simulink model "model_new_visual"  (R2023a)
settings: Solver=VariableStepAuto  StartTime=0.0  StopTime=3  RelTol=1e-3
model workspace: external: MATLAB File model_new_DataFile.m (data not in the file)
values from neighbouring files (symbols this model uses):
  smiData = struct    [model_new_DataFile.m]
undefined symbols (not defined in the file or in its folder): _, ____, ____16, ____19, ____20, ____3, ____4, ____4X6X3, ____6, ____6X10X3, ____7X11X2, ______, ______1, ______2, ______3_________________________, _______1_________________________2_________________________________航发支架总装, ________, ________1, ________20__1____6, ________6, _________, __________, __________2, __________40160, __________6x16x5, ____________, ____________2, ____________3X1, ______________, ______________1X5, __________________, ___________________, ____________________20__26____4, ____________________25__25____5, __________________SULERCH, ______________A, __________A, __________B, ______A__6, _X2_4E1D6746_X0_, _X2_652F64915EA7_X0_, _X2_7535673A5B8988C5677F_X0_, _X2_8F74627F677F_X0_, _航发支架总装, _默认_sldprt, A25, a__________100, BZ, C, CONNECTOR_5MMCLOSED2PIN_MALE_1, D1, DIP_SWITCH_8PIN_VIC2_1, DYJN, EC, EE, FUS606_REF_1, GE4C, IPOS__________, LAF30, M3________ ... (+34)
libraries: sm_lib x987, nesl_utility x6, simulink x4
(part 18 of 18)

== system model_new_visual/x__25_07_22_V1_STEP_1_RIGID/Subsystem/x__25_07_22_V1_STEP_1_RIGID1/CL3J_EC503_3D_25_07_22_V1_STEP_1_RIGID/PCB_ASM_4_ASM25_07_22_V1_STEP_1_RIGID/x5PIN_MINIUSB_SOCKET_1_1_125_07_22_V1_STEP_1_RIGID ==
  ReferenceFrame : sm_lib/Frames and Transforms/Reference Frame
  Solid : sm_lib/Body Elements/File Solid  ExtGeomFileName=5PIN_MINIUSB_SOCKET_1_1_1(25.07.22)-V1.STEP_默认_sldprt.STEP  UnitType=FromFile  ExtGeomFileUnits=m  StepReaderType=HEX  ExportConvexHullGeometry=off  InertiaType=Custom  Mass=smiData.Solid(76).mass  MassUnits=kg  CenterOfMass=smiData.Solid(76).CoM  CenterOfMassUnits=mm  MomentsOfInertia=smiData.Solid(76).MoI  MomentsOfInertiaUnits=kg*mm^2  ProductsOfInertia=smiData.Solid(76).PoI  ProductsOfInertiaUnits=kg*mm^2  BasedOnType=DensityFromFile  Density=1000  DensityUnits=kg/m^3  DoExposeReferenceFrame=on  SerializedFrames=<Frames/>  GraphicType=FromGeometry  MarkerShape=Sphere  MarkerSize=10  GraphicVisPropType=SimpleVisualProperties  GraphicDiffuseColor=smiData.Solid(76).color  GraphicSpecularColor=[0.5 0.5 0.5 1.0]  GraphicAmbientColor=[0.15 0.15 0.15 1.0]  GraphicEmissiveColor=[0.0 0.0 0.0 1.0]  GraphicShininess=75  GraphicOpacity=smiData.Solid(76).opacity
  F : PMIOPort  Side=Left
  connections:
  Solid/RConn1 -- ReferenceFrame/RConn1 -- F/RConn1

== system model_new_visual/x__25_07_22_V1_STEP_1_RIGID/Subsystem/x__25_07_22_V1_STEP_1_RIGID1/CL3J_EC503_3D_25_07_22_V1_STEP_1_RIGID/PCB_ASM_4_ASM25_07_22_V1_STEP_1_RIGID/FCI_USB_ANY_1_ASM25_07_22_V1_STEP_1_RIGID/MANIFOLD_SOLID_BREP_6679525_07_22_V1_STEP_1_RIGID ==
  ReferenceFrame : sm_lib/Frames and Transforms/Reference Frame
  Solid : sm_lib/Body Elements/File Solid  ExtGeomFileName=MANIFOLD_SOLID_BREP_66795(25.07.22)-V1.STEP_默认_sldprt.STEP  UnitType=FromFile  ExtGeomFileUnits=m  StepReaderType=HEX  ExportConvexHullGeometry=off  InertiaType=Custom  Mass=smiData.Solid(79).mass  MassUnits=kg  CenterOfMass=smiData.Solid(79).CoM  CenterOfMassUnits=mm  MomentsOfInertia=smiData.Solid(79).MoI  MomentsOfInertiaUnits=kg*mm^2  ProductsOfInertia=smiData.Solid(79).PoI  ProductsOfInertiaUnits=kg*mm^2  BasedOnType=DensityFromFile  Density=1000  DensityUnits=kg/m^3  DoExposeReferenceFrame=on  SerializedFrames=<Frames/>  GraphicType=FromGeometry  MarkerShape=Sphere  MarkerSize=10  GraphicVisPropType=SimpleVisualProperties  GraphicDiffuseColor=smiData.Solid(79).color  GraphicSpecularColor=[0.5 0.5 0.5 1.0]  GraphicAmbientColor=[0.15 0.15 0.15 1.0]  GraphicEmissiveColor=[0.0 0.0 0.0 1.0]  GraphicShininess=75  GraphicOpacity=smiData.Solid(79).opacity
  F : PMIOPort  Side=Left
  connections:
  Solid/RConn1 -- ReferenceFrame/RConn1 -- F/RConn1

== system model_new_visual/x__25_07_22_V1_STEP_1_RIGID/Subsystem/x__25_07_22_V1_STEP_1_RIGID1/CL3J_EC503_3D_25_07_22_V1_STEP_1_RIGID/PCB_ASM_4_ASM25_07_22_V1_STEP_1_RIGID/FCI_USB_ANY_1_ASM25_07_22_V1_STEP_1_RIGID/MANIFOLD_SOLID_BREP_6688325_07_22_V1_STEP_1_RIGID ==
  ReferenceFrame : sm_lib/Frames and Transforms/Reference Frame
  Solid : sm_lib/Body Elements/File Solid  ExtGeomFileName=MANIFOLD_SOLID_BREP_66883(25.07.22)-V1.STEP_默认_sldprt.STEP  UnitType=FromFile  ExtGeomFileUnits=m  StepReaderType=HEX  ExportConvexHullGeometry=off  InertiaType=Custom  Mass=smiData.Solid(78).mass  MassUnits=kg  CenterOfMass=smiData.Solid(78).CoM  CenterOfMassUnits=mm  MomentsOfInertia=smiData.Solid(78).MoI  MomentsOfInertiaUnits=kg*mm^2  ProductsOfInertia=smiData.Solid(78).PoI  ProductsOfInertiaUnits=kg*mm^2  BasedOnType=DensityFromFile  Density=1000  DensityUnits=kg/m^3  DoExposeReferenceFrame=on  SerializedFrames=<Frames/>  GraphicType=FromGeometry  MarkerShape=Sphere  MarkerSize=10  GraphicVisPropType=SimpleVisualProperties  GraphicDiffuseColor=smiData.Solid(78).color  GraphicSpecularColor=[0.5 0.5 0.5 1.0]  GraphicAmbientColor=[0.15 0.15 0.15 1.0]  GraphicEmissiveColor=[0.0 0.0 0.0 1.0]  GraphicShininess=75  GraphicOpacity=smiData.Solid(78).opacity
  F : PMIOPort  Side=Left
  connections:
  Solid/RConn1 -- ReferenceFrame/RConn1 -- F/RConn1

== system model_new_visual/x__25_07_22_V1_STEP_1_RIGID/Subsystem/x__25_07_22_V1_STEP_1_RIGID1/CL3J_EC503_3D_25_07_22_V1_STEP_1_RIGID/PCB_ASM_4_ASM25_07_22_V1_STEP_1_RIGID/x15EDGRHB_THR_3_5_10_1_ASM25_07_22_V1_STEP_1_RIGID/MANIFOLD_SOLID_BREP_11810025_07_22_V1_STEP_1_RIGID ==
  ReferenceFrame : sm_lib/Frames and Transforms/Reference Frame
  Solid : sm_lib/Body Elements/File Solid  ExtGeomFileName=MANIFOLD_SOLID_BREP_118100(25.07.22)-V1.STEP_默认_sldprt.STEP  UnitType=FromFile  ExtGeomFileUnits=m  StepReaderType=HEX  ExportConvexHullGeometry=off  InertiaType=Custom  Mass=smiData.Solid(82).mass  MassUnits=kg  CenterOfMass=smiData.Solid(82).CoM  CenterOfMassUnits=mm  MomentsOfInertia=smiData.Solid(82).MoI  MomentsOfInertiaUnits=kg*mm^2  ProductsOfInertia=smiData.Solid(82).PoI  ProductsOfInertiaUnits=kg*mm^2  BasedOnType=DensityFromFile  Density=1000  DensityUnits=kg/m^3  DoExposeReferenceFrame=on  SerializedFrames=<Frames/>  GraphicType=FromGeometry  MarkerShape=Sphere  MarkerSize=10  GraphicVisPropType=SimpleVisualProperties  GraphicDiffuseColor=smiData.Solid(82).color  GraphicSpecularColor=[0.5 0.5 0.5 1.0]  GraphicAmbientColor=[0.15 0.15 0.15 1.0]  GraphicEmissiveColor=[0.0 0.0 0.0 1.0]  GraphicShininess=75  GraphicOpacity=smiData.Solid(82).opacity
  F : PMIOPort  Side=Left
  connections:
  Solid/RConn1 -- ReferenceFrame/RConn1 -- F/RConn1

== system model_new_visual/x__25_07_22_V1_STEP_1_RIGID/Subsystem/x__25_07_22_V1_STEP_1_RIGID1/CL3J_EC503_3D_25_07_22_V1_STEP_1_RIGID/PCB_ASM_4_ASM25_07_22_V1_STEP_1_RIGID/x15EDGRHB_THR_3_5_10_1_ASM25_07_22_V1_STEP_1_RIGID/MANIFOLD_SOLID_BREP_11834725_07_22_V1_STEP_1_RIGID ==
  ReferenceFrame : sm_lib/Frames and Transforms/Reference Frame
  Solid : sm_lib/Body Elements/File Solid  ExtGeomFileName=MANIFOLD_SOLID_BREP_118347(25.07.22)-V1.STEP_默认_sldprt.STEP  UnitType=FromFile  ExtGeomFileUnits=m  StepReaderType=HEX  ExportConvexHullGeometry=off  InertiaType=Custom  Mass=smiData.Solid(83).mass  MassUnits=kg  CenterOfMass=smiData.Solid(83).CoM  CenterOfMassUnits=mm  MomentsOfInertia=smiData.Solid(83).MoI  MomentsOfInertiaUnits=kg*mm^2  ProductsOfInertia=smiData.Solid(83).PoI  ProductsOfInertiaUnits=kg*mm^2  BasedOnType=DensityFromFile  Density=1000  DensityUnits=kg/m^3  DoExposeReferenceFrame=on  SerializedFrames=<Frames/>  GraphicType=FromGeometry  MarkerShape=Sphere  MarkerSize=10  GraphicVisPropType=SimpleVisualProperties  GraphicDiffuseColor=smiData.Solid(83).color  GraphicSpecularColor=[0.5 0.5 0.5 1.0]  GraphicAmbientColor=[0.15 0.15 0.15 1.0]  GraphicEmissiveColor=[0.0 0.0 0.0 1.0]  GraphicShininess=75  GraphicOpacity=smiData.Solid(83).opacity
  F : PMIOPort  Side=Left
  connections:
  Solid/RConn1 -- ReferenceFrame/RConn1 -- F/RConn1

== system model_new_visual/x__25_07_22_V1_STEP_1_RIGID/Subsystem/x__25_07_22_V1_STEP_1_RIGID1/CL3J_EC503_3D_25_07_22_V1_STEP_1_RIGID/PCB_ASM_4_ASM25_07_22_V1_STEP_1_RIGID/x15EDGRHB_THR_3_5_10_1_ASM25_07_22_V1_STEP_1_RIGID/MANIFOLD_SOLID_BREP_11859425_07_22_V1_STEP_1_RIGID ==
  ReferenceFrame : sm_lib/Frames and Transforms/Reference Frame
  Solid : sm_lib/Body Elements/File Solid  ExtGeomFileName=MANIFOLD_SOLID_BREP_118594(25.07.22)-V1.STEP_默认_sldprt.STEP  UnitType=FromFile  ExtGeomFileUnits=m  StepReaderType=HEX  ExportConvexHullGeometry=off  InertiaType=Custom  Mass=smiData.Solid(85).mass  MassUnits=kg  CenterOfMass=smiData.Solid(85).CoM  CenterOfMassUnits=mm  MomentsOfInertia=smiData.Solid(85).MoI  MomentsOfInertiaUnits=kg*mm^2  ProductsOfInertia=smiData.Solid(85).PoI  ProductsOfInertiaUnits=kg*mm^2  BasedOnType=DensityFromFile  Density=1000  DensityUnits=kg/m^3  DoExposeReferenceFrame=on  SerializedFrames=<Frames/>  GraphicType=FromGeometry  MarkerShape=Sphere  MarkerSize=10  GraphicVisPropType=SimpleVisualProperties  GraphicDiffuseColor=smiData.Solid(85).color  GraphicSpecularColor=[0.5 0.5 0.5 1.0]  GraphicAmbientColor=[0.15 0.15 0.15 1.0]  GraphicEmissiveColor=[0.0 0.0 0.0 1.0]  GraphicShininess=75  GraphicOpacity=smiData.Solid(85).opacity
  F : PMIOPort  Side=Left
  connections:
  Solid/RConn1 -- ReferenceFrame/RConn1 -- F/RConn1

== system model_new_visual/x__25_07_22_V1_STEP_1_RIGID/Subsystem/x__25_07_22_V1_STEP_1_RIGID1/CL3J_EC503_3D_25_07_22_V1_STEP_1_RIGID/PCB_ASM_4_ASM25_07_22_V1_STEP_1_RIGID/x15EDGRHB_THR_3_5_10_1_ASM25_07_22_V1_STEP_1_RIGID/MANIFOLD_SOLID_BREP_11884125_07_22_V1_STEP_1_RIGID ==
  ReferenceFrame : sm_lib/Frames and Transforms/Reference Frame
  Solid : sm_lib/Body Elements/File Solid  ExtGeomFileName=MANIFOLD_SOLID_BREP_118841(25.07.22)-V1.STEP_默认_sldprt.STEP  UnitType=FromFile  ExtGeomFileUnits=m  StepReaderType=HEX  ExportConvexHullGeometry=off  InertiaType=Custom  Mass=smiData.Solid(81).mass  MassUnits=kg  CenterOfMass=smiData.Solid(81).CoM  CenterOfMassUnits=mm  MomentsOfInertia=smiData.Solid(81).MoI  MomentsOfInertiaUnits=kg*mm^2  ProductsOfInertia=smiData.Solid(81).PoI  ProductsOfInertiaUnits=kg*mm^2  BasedOnType=DensityFromFile  Density=1000  DensityUnits=kg/m^3  DoExposeReferenceFrame=on  SerializedFrames=<Frames/>  GraphicType=FromGeometry  MarkerShape=Sphere  MarkerSize=10  GraphicVisPropType=SimpleVisualProperties  GraphicDiffuseColor=smiData.Solid(81).color  GraphicSpecularColor=[0.5 0.5 0.5 1.0]  GraphicAmbientColor=[0.15 0.15 0.15 1.0]  GraphicEmissiveColor=[0.0 0.0 0.0 1.0]  GraphicShininess=75  GraphicOpacity=smiData.Solid(81).opacity
  F : PMIOPort  Side=Left
  connections:
  Solid/RConn1 -- ReferenceFrame/RConn1 -- F/RConn1

== system model_new_visual/x__25_07_22_V1_STEP_1_RIGID/Subsystem/x__25_07_22_V1_STEP_1_RIGID1/CL3J_EC503_3D_25_07_22_V1_STEP_1_RIGID/PCB_ASM_4_ASM25_07_22_V1_STEP_1_RIGID/x15EDGRHB_THR_3_5_10_1_ASM25_07_22_V1_STEP_1_RIGID/MANIFOLD_SOLID_BREP_11908825_07_22_V1_STEP_1_RIGID ==
  ReferenceFrame : sm_lib/Frames and Transforms/Reference Frame
  Solid : sm_lib/Body Elements/File Solid  ExtGeomFileName=MANIFOLD_SOLID_BREP_119088(25.07.22)-V1.STEP_默认_sldprt.STEP  UnitType=FromFile  ExtGeomFileUnits=m  StepReaderType=HEX  ExportConvexHullGeometry=off  InertiaType=Custom  Mass=smiData.Solid(84).mass  MassUnits=kg  CenterOfMass=smiData.Solid(84).CoM  CenterOfMassUnits=mm  MomentsOfInertia=smiData.Solid(84).MoI  MomentsOfInertiaUnits=kg*mm^2  ProductsOfInertia=smiData.Solid(84).PoI  ProductsOfInertiaUnits=kg*mm^2  BasedOnType=DensityFromFile  Density=1000  DensityUnits=kg/m^3  DoExposeReferenceFrame=on  SerializedFrames=<Frames/>  GraphicType=FromGeometry  MarkerShape=Sphere  MarkerSize=10  GraphicVisPropType=SimpleVisualProperties  GraphicDiffuseColor=smiData.Solid(84).color  GraphicSpecularColor=[0.5 0.5 0.5 1.0]  GraphicAmbientColor=[0.15 0.15 0.15 1.0]  GraphicEmissiveColor=[0.0 0.0 0.0 1.0]  GraphicShininess=75  GraphicOpacity=smiData.Solid(84).opacity
  F : PMIOPort  Side=Left
  connections:
  Solid/RConn1 -- ReferenceFrame/RConn1 -- F/RConn1

== system model_new_visual/x__25_07_22_V1_STEP_1_RIGID/Subsystem/x__25_07_22_V1_STEP_1_RIGID1/CL3J_EC503_3D_25_07_22_V1_STEP_1_RIGID/PCB_ASM_4_ASM25_07_22_V1_STEP_1_RIGID/x15EDGRHB_THR_3_5_10_1_ASM25_07_22_V1_STEP_1_RIGID/MANIFOLD_SOLID_BREP_11933525_07_22_V1_STEP_1_RIGID ==
  ReferenceFrame : sm_lib/Frames and Transforms/Reference Frame
  Solid : sm_lib/Body Elements/File Solid  ExtGeomFileName=MANIFOLD_SOLID_BREP_119335(25.07.22)-V1.STEP_默认_sldprt.STEP  UnitType=FromFile  ExtGeomFileUnits=m  StepReaderType=HEX  ExportConvexHullGeometry=off  InertiaType=Custom  Mass=smiData.Solid(80).mass  MassUnits=kg  CenterOfMass=smiData.Solid(80).CoM  CenterOfMassUnits=mm  MomentsOfInertia=smiData.Solid(80).MoI  MomentsOfInertiaUnits=kg*mm^2  ProductsOfInertia=smiData.Solid(80).PoI  ProductsOfInertiaUnits=kg*mm^2  BasedOnType=DensityFromFile  Density=1000  DensityUnits=kg/m^3  DoExposeReferenceFrame=on  SerializedFrames=<Frames/>  GraphicType=FromGeometry  MarkerShape=Sphere  MarkerSize=10  GraphicVisPropType=SimpleVisualProperties  GraphicDiffuseColor=smiData.Solid(80).color  GraphicSpecularColor=[0.5 0.5 0.5 1.0]  GraphicAmbientColor=[0.15 0.15 0.15 1.0]  GraphicEmissiveColor=[0.0 0.0 0.0 1.0]  GraphicShininess=75  GraphicOpacity=smiData.Solid(80).opacity
  F : PMIOPort  Side=Left
  connections:
  Solid/RConn1 -- ReferenceFrame/RConn1 -- F/RConn1

== system model_new_visual/x__25_07_22_V1_STEP_1_RIGID/Subsystem/x__25_07_22_V1_STEP_1_RIGID1/CL3J_EC503_3D_25_07_22_V1_STEP_1_RIGID/PCB_ASM_4_ASM25_07_22_V1_STEP_1_RIGID/x15EDGRHB_THR_3_5_10_1_ASM25_07_22_V1_STEP_1_RIGID/MANIFOLD_SOLID_BREP_11958225_07_22_V1_STEP_1_RIGID ==
  ReferenceFrame : sm_lib/Frames and Transforms/Reference Frame
  Solid : sm_lib/Body Elements/File Solid  ExtGeomFileName=MANIFOLD_SOLID_BREP_119582(25.07.22)-V1.STEP_默认_sldprt.STEP  UnitType=FromFile  ExtGeomFileUnits=m  StepReaderType=HEX  ExportConvexHullGeometry=off  InertiaType=Custom  Mass=smiData.Solid(90).mass  MassUnits=kg  CenterOfMass=smiData.Solid(90).CoM  CenterOfMassUnits=mm  MomentsOfInertia=smiData.Solid(90).MoI  MomentsOfInertiaUnits=kg*mm^2  ProductsOfInertia=smiData.Solid(90).PoI  ProductsOfInertiaUnits=kg*mm^2  BasedOnType=DensityFromFile  Density=1000  DensityUnits=kg/m^3  DoExposeReferenceFrame=on  SerializedFrames=<Frames/>  GraphicType=FromGeometry  MarkerShape=Sphere  MarkerSize=10  GraphicVisPropType=SimpleVisualProperties  GraphicDiffuseColor=smiData.Solid(90).color  GraphicSpecularColor=[0.5 0.5 0.5 1.0]  GraphicAmbientColor=[0.15 0.15 0.15 1.0]  GraphicEmissiveColor=[0.0 0.0 0.0 1.0]  GraphicShininess=75  GraphicOpacity=smiData.Solid(90).opacity
  F : PMIOPort  Side=Left
  connections:
  Solid/RConn1 -- ReferenceFrame/RConn1 -- F/RConn1

== system model_new_visual/x__25_07_22_V1_STEP_1_RIGID/Subsystem/x__25_07_22_V1_STEP_1_RIGID1/CL3J_EC503_3D_25_07_22_V1_STEP_1_RIGID/PCB_ASM_4_ASM25_07_22_V1_STEP_1_RIGID/x15EDGRHB_THR_3_5_10_1_ASM25_07_22_V1_STEP_1_RIGID/MANIFOLD_SOLID_BREP_11982925_07_22_V1_STEP_1_RIGID ==
  ReferenceFrame : sm_lib/Frames and Transforms/Reference Frame
  Solid : sm_lib/Body Elements/File Solid  ExtGeomFileName=MANIFOLD_SOLID_BREP_119829(25.07.22)-V1.STEP_默认_sldprt.STEP  UnitType=FromFile  ExtGeomFileUnits=m  StepReaderType=HEX  ExportConvexHullGeometry=off  InertiaType=Custom  Mass=smiData.Solid(89).mass  MassUnits=kg  CenterOfMass=smiData.Solid(89).CoM  CenterOfMassUnits=mm  MomentsOfInertia=smiData.Solid(89).MoI  MomentsOfInertiaUnits=kg*mm^2  ProductsOfInertia=smiData.Solid(89).PoI  ProductsOfInertiaUnits=kg*mm^2  BasedOnType=DensityFromFile  Density=1000  DensityUnits=kg/m^3  DoExposeReferenceFrame=on  SerializedFrames=<Frames/>  GraphicType=FromGeometry  MarkerShape=Sphere  MarkerSize=10  GraphicVisPropType=SimpleVisualProperties  GraphicDiffuseColor=smiData.Solid(89).color  GraphicSpecularColor=[0.5 0.5 0.5 1.0]  GraphicAmbientColor=[0.15 0.15 0.15 1.0]  GraphicEmissiveColor=[0.0 0.0 0.0 1.0]  GraphicShininess=75  GraphicOpacity=smiData.Solid(89).opacity
  F : PMIOPort  Side=Left
  connections:
  Solid/RConn1 -- ReferenceFrame/RConn1 -- F/RConn1

== system model_new_visual/x__25_07_22_V1_STEP_1_RIGID/Subsystem/x__25_07_22_V1_STEP_1_RIGID1/CL3J_EC503_3D_25_07_22_V1_STEP_1_RIGID/PCB_ASM_4_ASM25_07_22_V1_STEP_1_RIGID/x15EDGRHB_THR_3_5_10_1_ASM25_07_22_V1_STEP_1_RIGID/MANIFOLD_SOLID_BREP_12007625_07_22_V1_STEP_1_RIGID ==
  ReferenceFrame : sm_lib/Frames and Transforms/Reference Frame
  Solid : sm_lib/Body Elements/File Solid  ExtGeomFileName=MANIFOLD_SOLID_BREP_120076(25.07.22)-V1.STEP_默认_sldprt.STEP  UnitType=FromFile  ExtGeomFileUnits=m  StepReaderType=HEX  ExportConvexHullGeometry=off  InertiaType=Custom  Mass=smiData.Solid(87).mass  MassUnits=kg  CenterOfMass=smiData.Solid(87).CoM  CenterOfMassUnits=mm  MomentsOfInertia=smiData.Solid(87).MoI  MomentsOfInertiaUnits=kg*mm^2  ProductsOfInertia=smiData.Solid(87).PoI  ProductsOfInertiaUnits=kg*mm^2  BasedOnType=DensityFromFile  Density=1000  DensityUnits=kg/m^3  DoExposeReferenceFrame=on  SerializedFrames=<Frames/>  GraphicType=FromGeometry  MarkerShape=Sphere  MarkerSize=10  GraphicVisPropType=SimpleVisualProperties  GraphicDiffuseColor=smiData.Solid(87).color  GraphicSpecularColor=[0.5 0.5 0.5 1.0]  GraphicAmbientColor=[0.15 0.15 0.15 1.0]  GraphicEmissiveColor=[0.0 0.0 0.0 1.0]  GraphicShininess=75  GraphicOpacity=smiData.Solid(87).opacity
  F : PMIOPort  Side=Left
  connections:
  Solid/RConn1 -- ReferenceFrame/RConn1 -- F/RConn1

== system model_new_visual/x__25_07_22_V1_STEP_1_RIGID/Subsystem/x__25_07_22_V1_STEP_1_RIGID1/CL3J_EC503_3D_25_07_22_V1_STEP_1_RIGID/PCB_ASM_4_ASM25_07_22_V1_STEP_1_RIGID/x15EDGRHB_THR_3_5_10_1_ASM25_07_22_V1_STEP_1_RIGID/MANIFOLD_SOLID_BREP_12032325_07_22_V1_STEP_1_RIGID ==
  ReferenceFrame : sm_lib/Frames and Transforms/Reference Frame
  Solid : sm_lib/Body Elements/File Solid  ExtGeomFileName=MANIFOLD_SOLID_BREP_120323(25.07.22)-V1.STEP_默认_sldprt.STEP  UnitType=FromFile  ExtGeomFileUnits=m  StepReaderType=HEX  ExportConvexHullGeometry=off  InertiaType=Custom  Mass=smiData.Solid(86).mass  MassUnits=kg  CenterOfMass=smiData.Solid(86).CoM  CenterOfMassUnits=mm  MomentsOfInertia=smiData.Solid(86).MoI  MomentsOfInertiaUnits=kg*mm^2  ProductsOfInertia=smiData.Solid(86).PoI  ProductsOfInertiaUnits=kg*mm^2  BasedOnType=DensityFromFile  Density=1000  DensityUnits=kg/m^3  DoExposeReferenceFrame=on  SerializedFrames=<Frames/>  GraphicType=FromGeometry  MarkerShape=Sphere  MarkerSize=10  GraphicVisPropType=SimpleVisualProperties  GraphicDiffuseColor=smiData.Solid(86).color  GraphicSpecularColor=[0.5 0.5 0.5 1.0]  GraphicAmbientColor=[0.15 0.15 0.15 1.0]  GraphicEmissiveColor=[0.0 0.0 0.0 1.0]  GraphicShininess=75  GraphicOpacity=smiData.Solid(86).opacity
  F : PMIOPort  Side=Left
  connections:
  Solid/RConn1 -- ReferenceFrame/RConn1 -- F/RConn1

== system model_new_visual/x__25_07_22_V1_STEP_1_RIGID/Subsystem/x__25_07_22_V1_STEP_1_RIGID1/CL3J_EC503_3D_25_07_22_V1_STEP_1_RIGID/PCB_ASM_4_ASM25_07_22_V1_STEP_1_RIGID/x15EDGRHB_THR_3_5_10_1_ASM25_07_22_V1_STEP_1_RIGID/MANIFOLD_SOLID_BREP_12057025_07_22_V1_STEP_1_RIGID ==
  ReferenceFrame : sm_lib/Frames and Transforms/Reference Frame
  Solid : sm_lib/Body Elements/File Solid  ExtGeomFileName=MANIFOLD_SOLID_BREP_120570(25.07.22)-V1.STEP_默认_sldprt.STEP  UnitType=FromFile  ExtGeomFileUnits=m  StepReaderType=HEX  ExportConvexHullGeometry=off  InertiaType=Custom  Mass=smiData.Solid(88).mass  MassUnits=kg  CenterOfMass=smiData.Solid(88).CoM  CenterOfMassUnits=mm  MomentsOfInertia=smiData.Solid(88).MoI  MomentsOfInertiaUnits=kg*mm^2  ProductsOfInertia=smiData.Solid(88).PoI  ProductsOfInertiaUnits=kg*mm^2  BasedOnType=DensityFromFile  Density=1000  DensityUnits=kg/m^3  DoExposeReferenceFrame=on  SerializedFrames=<Frames/>  GraphicType=FromGeometry  MarkerShape=Sphere  MarkerSize=10  GraphicVisPropType=SimpleVisualProperties  GraphicDiffuseColor=smiData.Solid(88).color  GraphicSpecularColor=[0.5 0.5 0.5 1.0]  GraphicAmbientColor=[0.15 0.15 0.15 1.0]  GraphicEmissiveColor=[0.0 0.0 0.0 1.0]  GraphicShininess=75  GraphicOpacity=smiData.Solid(88).opacity
  F : PMIOPort  Side=Left
  connections:
  Solid/RConn1 -- ReferenceFrame/RConn1 -- F/RConn1
